simulink model "G474_Mode2_Direct_Start"  (R2024b)
settings: Solver=FixedStepDiscrete  StartTime=0.0  StopTime=q.stop_time  FixedStep=p.Ts  RelTol=1e-3
InitFcn:
  | m2_project_root=fileparts(fileparts(get_param(bdroot,'FileName')));Simulink.fileGenControl('set','CacheFolder',fullfile(m2_project_root,'work'),'CodeGenFolder',fullfile(m2_project_root,'work'),'createDir',true);
model workspace (MAT data in the model file):
  fSin = [0 0.00153398001567 0.00306795700453 0.00460192607716 0.00613588513806 0.00766982883215 0.00920375529677 0.0107376594096 0.0122715383768 0.0138053894043 0.0153392059729 0.0168729871511 ... (1025 elements, 1025x1)]
  p.Rs = 0.875
  p.Ls = 0.0002
  p.Ld = 0.0002
  p.Lq = 0.0002
  p.Flux = 0.00752
  p.MOTOR_POLES = 14
  p.Ts = 5e-05
  p.Gain = 5000
  p.PLL_BW_Hz = 15
  p.Comp_BW_Hz = 5
  p.PLL_kp = 188.495559215
  p.PLL_ki = 0.444132198049
  p.Comp_Kp = 62.8318530718
  p.Comp_Ki = 0.0493480220054
  p.Comp_Mode = 0
  p.SMO_Kslide = 10
  p.SMO_Boundary = 0.002
  p.V_deadtime = 0.3
  p.current_deadband = 0.01
  p.pll_step_limit = 0.157079632679
  p.speed_decimation = 8
  p.speed_filter_old = 0.95
  p.speed_filter_new = 0.05
  q.Ts = 5e-05
  q.Rs = 0.875
  q.Ld = 0.0002
  q.Lq = 0.0002
  q.Flux = 0.00752
  q.pole_pairs = 7
  q.target_rpm = 200
  q.second_rpm = 400
  q.third_rpm = 1000
  q.switch_1 = 0.8
  q.switch_2 = 1.6
  q.Vbus = 12
  q.stop_time = 4
  q.J = 2e-05
  q.B = 1e-05
  q.load_torque = 0.005
  q.initial_theta_e = 0.523598775598
  q.initial_rpm = 0
  q.actual_deadtime_V = 0.3
  q.speed_iq_sign = -1
  q.ramp_step = 0.05
  q.current_channel_sign = 1
  q.initial_state = [0; 0; 0; 0.523598775598]
  s0.psi_s = [0; 0]
  s0.theta = 0
(part 1 of 2)
settings Model: Creator=QXZ-030079  LastModifiedBy=QXZ-030079
settings DataIOCC: SignalLogging=off

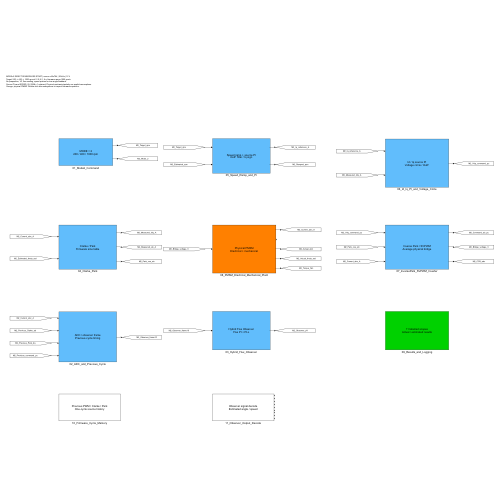
[thumbnail: Simulink's stored preview of the top-level diagram]
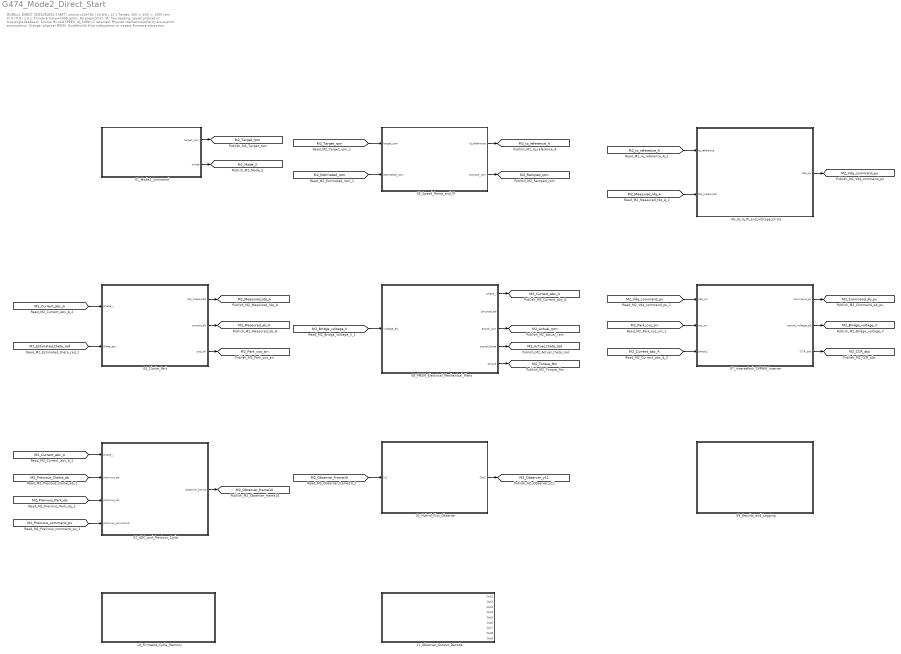
== system G474_Mode2_Direct_Start ==
  note: MODE=2 DIRECT SENSORLESS START | source c43e794 | 20 kHz | 12 V
      | Target: 200 -> 400 -> 1000 rpm at 0 / 0.8 / 1.6 s; firmware ramp=1000 rpm/s.
      | No preposition, VF, flux seeding, speed preload or true-angle feedback.
      | Source PIs and SPEED_IQ_SIGN=-1 retained. Physical mechanics/polarity are explicit assumptions.
      | Orange: physical PMSM. Double-click blue subsystems to inspect firmware equations.
  01_Mode2_Command : Subsystem
      mask Display: disp('MODE = 2\n200 / 400 / 1000 rpm');
  02_ADC_and_Previous_Cycle : Subsystem
      mask Display: disp('ADC / observer frame\nPrevious-cycle timing');
  03_Hybrid_Flux_Observer : Subsystem
      settings: OpenFcn=open_system(gcb,'force')
      mask Display: disp('Hybrid Flux Observer\nFlux PI + PLL');
  04_Clarke_Park : Subsystem
      mask Display: disp('Clarke / Park\nFirmware sine table');
  05_Speed_Ramp_and_PI : Subsystem
      mask Display: disp('Speed ramp + source PI\nOutF filter / Iq sign');
  06_Id_Iq_PI_and_Voltage_Circle : Subsystem
      mask Display: disp('Id / Iq source PI\nVoltage circle / OutF');
  07_InversePark_SVPWM_Inverter : Subsystem
      mask Display: disp('Inverse Park / SVPWM\nAverage physical bridge');
  08_PMSM_Electrical_Mechanical_Plant : Subsystem
      mask Display: disp('Physical PMSM\nElectrical + mechanical');
  09_Results_and_Logging : Subsystem
      mask Display: disp('11 labelled scopes\nActual / estimated results');
  10_Firmware_Cycle_Memory : Subsystem
      mask Display: disp('Previous PWM / Clarke / Park\nOne-cycle source history');
  11_Observer_Output_Decode : Subsystem
      mask Display: disp('Observer signal decode\nEstimated angle / speed');
  tag scope: M2_Actual_rpm=global, M2_Actual_theta_rad=global, M2_Bridge_voltage_V=global, M2_CCR_abc=global, M2_Command_ab_pu=global, M2_Current_abc_A=global, M2_Iq_reference_A=global, M2_Measured_Idq_A=global, M2_Measured_ab_A=global, M2_Mode_2=global, M2_Observer_frame10=global, M2_Observer_y11=global, M2_Park_cos_sin=global, M2_Ramped_rpm=global, M2_Target_rpm=global, M2_Torque_Nm=global, M2_Vdq_command_pu=global
  wires:
  01_Mode2_Command/2(mode) -> [M2_Mode_2]
  07_InversePark_SVPWM_Inverter/3(CCR_abc) -> [M2_CCR_abc]
  05_Speed_Ramp_and_PI/2(ramped_rpm) -> [M2_Ramped_rpm]
  08_PMSM_Electrical_Mechanical_Plant/5(torque) -> [M2_Torque_Nm]
  08_PMSM_Electrical_Mechanical_Plant/4(actual_theta) -> [M2_Actual_theta_rad]
  08_PMSM_Electrical_Mechanical_Plant/3(actual_rpm) -> [M2_Actual_rpm]
  07_InversePark_SVPWM_Inverter/2(actual_voltage_ab) -> [M2_Bridge_voltage_V]
  [M2_Bridge_voltage_V] -> 08_PMSM_Electrical_Mechanical_Plant/1(voltage_ab)
  04_Clarke_Park/3(cos_sin) -> [M2_Park_cos_sin]
  [M2_Park_cos_sin] -> 07_InversePark_SVPWM_Inverter/2(cos_sin)
  06_Id_Iq_PI_and_Voltage_Circle/1(Vdq_pu) -> [M2_Vdq_command_pu]
  [M2_Vdq_command_pu] -> 07_InversePark_SVPWM_Inverter/1(Vdq_pu)
  05_Speed_Ramp_and_PI/1(Iq_reference) -> [M2_Iq_reference_A]
  [M2_Iq_reference_A] -> 06_Id_Iq_PI_and_Voltage_Circle/1(Iq_reference)
  [M2_Estimated_rpm] -> 05_Speed_Ramp_and_PI/2(estimated_rpm)
  01_Mode2_Command/1(target_rpm) -> [M2_Target_rpm]
  [M2_Target_rpm] -> 05_Speed_Ramp_and_PI/1(target_rpm)
  [M2_Estimated_theta_rad] -> 04_Clarke_Park/2(theta_est)
  03_Hybrid_Flux_Observer/1(Out1) -> [M2_Observer_y11]
  02_ADC_and_Previous_Cycle/1(observer_frame) -> [M2_Observer_frame10]
  [M2_Observer_frame10] -> 03_Hybrid_Flux_Observer/1(In1)
  [M2_Previous_command_pu] -> 02_ADC_and_Previous_Cycle/4(previous_command)
  [M2_Previous_Park_dq] -> 02_ADC_and_Previous_Cycle/3(previous_dq)
  [M2_Previous_Clarke_ab] -> 02_ADC_and_Previous_Cycle/2(previous_ab)
  08_PMSM_Electrical_Mechanical_Plant/1(phase_i) -> [M2_Current_abc_A]
  [M2_Current_abc_A] -> 02_ADC_and_Previous_Cycle/1(phase_i)
  [M2_Current_abc_A] -> 04_Clarke_Park/1(phase_i)
  [M2_Current_abc_A] -> 07_InversePark_SVPWM_Inverter/3(phase_i)
  04_Clarke_Park/1(Idq_measured) -> [M2_Measured_Idq_A]
  [M2_Measured_Idq_A] -> 06_Id_Iq_PI_and_Voltage_Circle/2(Idq_measured)
  04_Clarke_Park/2(current_ab) -> [M2_Measured_ab_A]
  07_InversePark_SVPWM_Inverter/1(command_pu) -> [M2_Command_ab_pu]

== system G474_Mode2_Direct_Start/01_Mode2_Command ==
  Initial_200rpm : Constant  Value=q.target_rpm
  MODE_SENSORLESS_2 : Constant  Value=2
  Speed_schedule : Sum  Inputs=+++
  Switch_to_1000rpm : Step  Time=q.switch_2  After=q.third_rpm-q.second_rpm  SampleTime=p.Ts
  Switch_to_400rpm : Step  Time=q.switch_1  After=q.second_rpm-q.target_rpm  SampleTime=p.Ts
  target_rpm : Outport
  mode : Outport  Port=2
  wires:
  MODE_SENSORLESS_2/1 -> mode/1
  Speed_schedule/1 -> target_rpm/1
  Initial_200rpm/1 -> Speed_schedule/1
  Switch_to_400rpm/1 -> Speed_schedule/2
  Switch_to_1000rpm/1 -> Speed_schedule/3

== system G474_Mode2_Direct_Start/02_ADC_and_Previous_Cycle ==
  phase_i : Inport
  previous_ab : Inport  Port=2
  previous_dq : Inport  Port=3
  previous_command : Inport  Port=4
  Firmware_call_order : MATLAB Function  TreatAsAtomicUnit=on
  observer_frame : Outport
  wires:
  previous_command/1 -> Firmware_call_order/1(old_command)
  phase_i/1 -> Firmware_call_order/2(phase_i)
  previous_ab/1 -> Firmware_call_order/3(old_ab)
  previous_dq/1 -> Firmware_call_order/4(old_dq)
  Firmware_call_order/1(frame) -> observer_frame/1

== system G474_Mode2_Direct_Start/03_Hybrid_Flux_Observer ==
  In1 : Inport
  01_Voltage_Compensation : Subsystem
      settings: OpenFcn=open_system(gcb,'force')
      mask Display: port_label('input',1,'command_pu');port_label('input',2,'phase_current');port_label('input',3,'Vbus');port_label('input',4,'Km');port_label('output',1,'voltage_V');
  02_Active_Flux_Models : Subsystem
      settings: OpenFcn=open_system(gcb,'force')
      mask Display: port_label('input',1,'theta_previous');port_label('input',2,'current_ab');port_label('input',3,'psi_s_previous');port_label('input',4,'Id');port_label('output',1,'psi_I');port_label('output',2,'psi_V');
  03_Flux_Feedback : Subsystem
      settings: OpenFcn=open_system(gcb,'force')
      mask Display: port_label('input',1,'psi_I');port_label('input',2,'psi_V');port_label('output',1,'Ucomp');
  04_Stator_Integrator : Subsystem
      settings: OpenFcn=open_system(gcb,'force')
      mask Display: port_label('input',1,'voltage_V');port_label('input',2,'current_ab');port_label('input',3,'Ucomp');port_label('output',1,'psi_s_new');port_label('output',2,'psi_s_previous');
  05_PLL_and_Angle : Subsystem
      settings: OpenFcn=open_system(gcb,'force')
      mask Display: port_label('input',1,'psi_V');port_label('output',1,'theta_previous');port_label('output',2,'step_rad');port_label('output',3,'theta_new');port_label('output',4,'PLL_error');
  06_Speed_Filter : Subsystem
      settings: OpenFcn=open_system(gcb,'force')
      mask Display: port_label('input',1,'step_rad');port_label('output',1,'electrical_Hz');port_label('output',2,'firmware_RPM');
  Input split : Demux  Outputs=[2 3 2 1 1 1]
  Results : Mux  Inputs=8
  Out1 : Outport
  wires:
  03_Flux_Feedback/1(Ucomp) -> 04_Stator_Integrator/3(Ucomp)
  02_Active_Flux_Models/2(psi_V) -> 05_PLL_and_Angle/1(psi_V), Results/4, 03_Flux_Feedback/2(psi_V)
  06_Speed_Filter/2(firmware_RPM) -> Results/3
  06_Speed_Filter/1(electrical_Hz) -> Results/2
  Results/1 -> Out1/1
  04_Stator_Integrator/2(psi_s_previous) -> 02_Active_Flux_Models/3(psi_s_previous)
  04_Stator_Integrator/1(psi_s_new) -> Results/5
  05_PLL_and_Angle/4(PLL_error) -> Results/6
  05_PLL_and_Angle/3(theta_new) -> Results/1
  05_PLL_and_Angle/2(step_rad) -> 06_Speed_Filter/1(step_rad), Results/7
  01_Voltage_Compensation/1(voltage_V) -> 04_Stator_Integrator/1(voltage_V), Results/8
  Input split/5 -> 01_Voltage_Compensation/3(Vbus)
  02_Active_Flux_Models/1(psi_I) -> 03_Flux_Feedback/1(psi_I)
  Input split/6 -> 01_Voltage_Compensation/4(Km)
  Input split/3 -> 02_Active_Flux_Models/2(current_ab), 04_Stator_Integrator/2(current_ab)
  Input split/1 -> 01_Voltage_Compensation/1(command_pu)
  Input split/4 -> 02_Active_Flux_Models/4(Id)
  In1/1 -> Input split/1
  Input split/2 -> 01_Voltage_Compensation/2(phase_current)
  05_PLL_and_Angle/1(theta_previous) -> 02_Active_Flux_Models/1(theta_previous)

== system G474_Mode2_Direct_Start/04_Clarke_Park ==
  phase_i : Inport
  theta_est : Inport  Port=2
  Source_lookup_and_transform : MATLAB Function  TreatAsAtomicUnit=on
  Idq_measured : Outport
  current_ab : Outport  Port=2
  cos_sin : Outport  Port=3
  wires:
  phase_i/1 -> Source_lookup_and_transform/1(iabc)
  Source_lookup_and_transform/3(cs) -> cos_sin/1
  theta_est/1 -> Source_lookup_and_transform/2(theta)
  Source_lookup_and_transform/1(dq) -> Idq_measured/1
  Source_lookup_and_transform/2(iab) -> current_ab/1

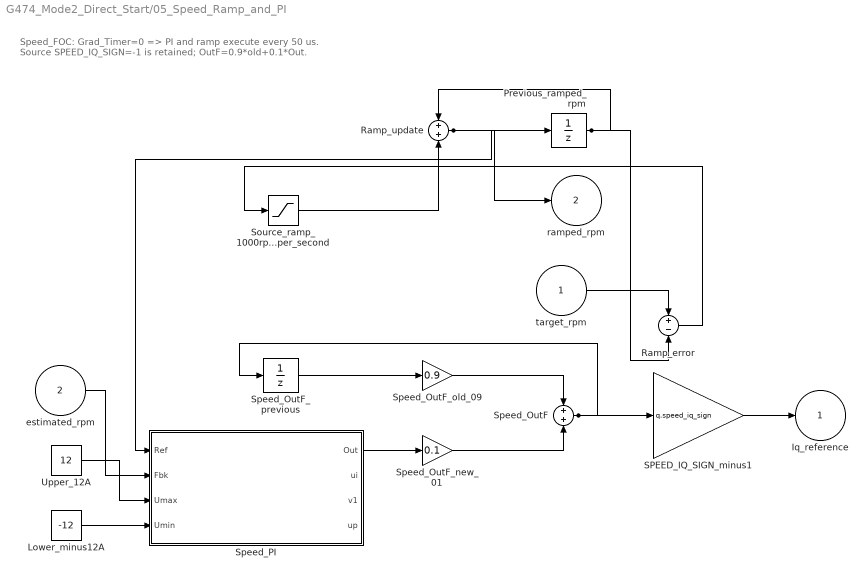
== system G474_Mode2_Direct_Start/05_Speed_Ramp_and_PI ==
  note: Speed_FOC: Grad_Timer=0 => PI and ramp execute every 50 us.
      | Source SPEED_IQ_SIGN=-1 is retained; OutF=0.9*old+0.1*Out.
  target_rpm : Inport
  estimated_rpm : Inport  Port=2
  Lower_minus12A : Constant  Value=-12
  Previous_ramped_rpm : UnitDelay  SampleTime=p.Ts  HasFrameUpgradeWarning=on
  Ramp_error : Sum  Inputs=+-
  Ramp_update : Sum
  SPEED_IQ_SIGN_minus1 : Gain  Gain=q.speed_iq_sign
  Source_ramp_1000rpm_per_second : Saturate  UpperLimit=q.ramp_step  LowerLimit=-q.ramp_step
  Speed_OutF : Sum
  Speed_OutF_new_01 : Gain  Gain=0.1
  Speed_OutF_old_09 : Gain  Gain=0.9
  Speed_OutF_previous : UnitDelay  SampleTime=p.Ts  HasFrameUpgradeWarning=on
  Speed_PI : Subsystem  mask{Kp=0.01, Ki=0.0001, Ts=p.Ts}
      mask prompts: Kp "Kp (source coefficient)"; Ki "Ki (per call, already discrete)"; Ts "Execution period (s)"
      settings: OpenFcn=open_system(gcb,'force')
      mask Display: port_label('input',1,'Ref');port_label('input',2,'Fbk');port_label('input',3,'Umax');port_label('input',4,'Umin');port_label('output',1,'Out');port_label('output',2,'ui');port_label('output',3,'v1');port_label('output',4,'up');
  Upper_12A : Constant  Value=12
  Iq_reference : Outport
  ramped_rpm : Outport  Port=2
  wires:
  Speed_OutF_old_09/1 -> Speed_OutF/1
  Ramp_update/1 -> Speed_PI/1(Ref), Previous_ramped_rpm/1, ramped_rpm/1
  Speed_PI/1(Out) -> Speed_OutF_new_01/1
  estimated_rpm/1 -> Speed_PI/2(Fbk)
  Upper_12A/1 -> Speed_PI/3(Umax)
  Source_ramp_1000rpm_per_second/1 -> Ramp_update/2
  Lower_minus12A/1 -> Speed_PI/4(Umin)
  Speed_OutF_previous/1 -> Speed_OutF_old_09/1
  target_rpm/1 -> Ramp_error/1
  Speed_OutF_new_01/1 -> Speed_OutF/2
  Previous_ramped_rpm/1 -> Ramp_error/2, Ramp_update/1
  Speed_OutF/1 -> Speed_OutF_previous/1, SPEED_IQ_SIGN_minus1/1
  Ramp_error/1 -> Source_ramp_1000rpm_per_second/1
  SPEED_IQ_SIGN_minus1/1 -> Iq_reference/1

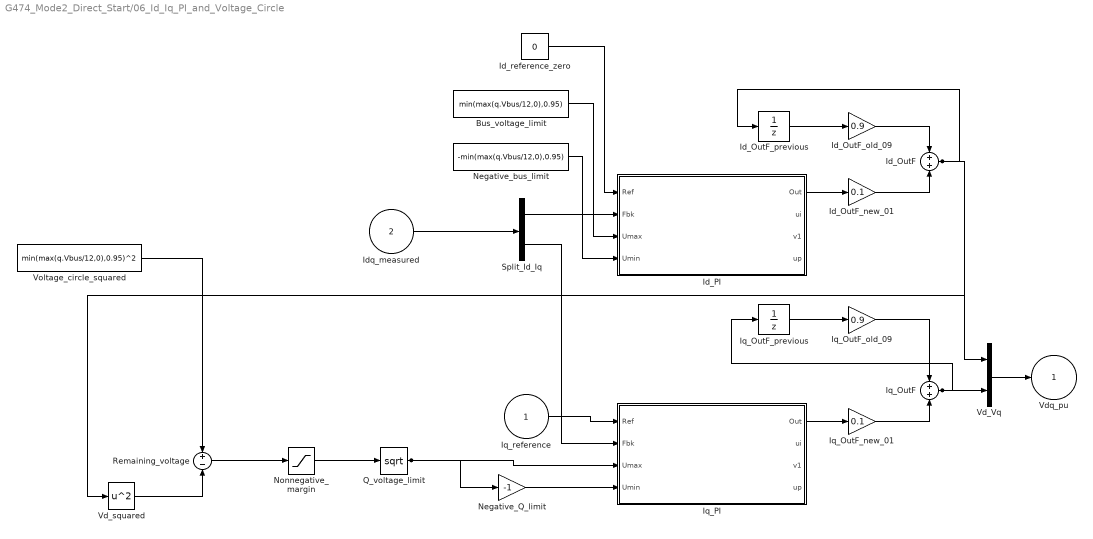
== system G474_Mode2_Direct_Start/06_Id_Iq_PI_and_Voltage_Circle ==
  Iq_reference : Inport
  Idq_measured : Inport  Port=2
  Bus_voltage_limit : Constant  Value=min(max(q.Vbus/12,0),0.95)
  Id_OutF : Sum
  Id_OutF_new_01 : Gain  Gain=0.1
  Id_OutF_old_09 : Gain  Gain=0.9
  Id_OutF_previous : UnitDelay  SampleTime=p.Ts  HasFrameUpgradeWarning=on
  Id_PI : Subsystem  mask{Kp=0.01, Ki=0.00001, Ts=p.Ts}
      mask prompts: Kp "Kp (source coefficient)"; Ki "Ki (per call, already discrete)"; Ts "Execution period (s)"
      settings: OpenFcn=open_system(gcb,'force')
      mask Display: port_label('input',1,'Ref');port_label('input',2,'Fbk');port_label('input',3,'Umax');port_label('input',4,'Umin');port_label('output',1,'Out');port_label('output',2,'ui');port_label('output',3,'v1');port_label('output',4,'up');
  Id_reference_zero : Constant  Value=0
  Iq_OutF : Sum
  Iq_OutF_new_01 : Gain  Gain=0.1
  Iq_OutF_old_09 : Gain  Gain=0.9
  Iq_OutF_previous : UnitDelay  SampleTime=p.Ts  HasFrameUpgradeWarning=on
  Iq_PI : Subsystem  mask{Kp=0.01, Ki=0.00001, Ts=p.Ts}
      mask prompts: Kp "Kp (source coefficient)"; Ki "Ki (per call, already discrete)"; Ts "Execution period (s)"
      settings: OpenFcn=open_system(gcb,'force')
      mask Display: port_label('input',1,'Ref');port_label('input',2,'Fbk');port_label('input',3,'Umax');port_label('input',4,'Umin');port_label('output',1,'Out');port_label('output',2,'ui');port_label('output',3,'v1');port_label('output',4,'up');
  Negative_Q_limit : Gain  Gain=-1
  Negative_bus_limit : Constant  Value=-min(max(q.Vbus/12,0),0.95)
  Nonnegative_margin : Saturate  UpperLimit=inf  LowerLimit=0
  Q_voltage_limit : Math  Operator=sqrt
  Remaining_voltage : Sum  Inputs=+-
  Split_Id_Iq : Demux  Outputs=2
  Vd_Vq : Mux  Inputs=2
  Vd_squared : Math  Operator=square
  Voltage_circle_squared : Constant  Value=min(max(q.Vbus/12,0),0.95)^2
  Vdq_pu : Outport
  wires:
  Id_reference_zero/1 -> Id_PI/1(Ref)
  Voltage_circle_squared/1 -> Remaining_voltage/1
  Remaining_voltage/1 -> Nonnegative_margin/1
  Iq_reference/1 -> Iq_PI/1(Ref)
  Vd_squared/1 -> Remaining_voltage/2
  Idq_measured/1 -> Split_Id_Iq/1
  Nonnegative_margin/1 -> Q_voltage_limit/1
  Q_voltage_limit/1 -> Iq_PI/3(Umax), Negative_Q_limit/1
  Bus_voltage_limit/1 -> Id_PI/3(Umax)
  Negative_bus_limit/1 -> Id_PI/4(Umin)
  Split_Id_Iq/1 -> Id_PI/2(Fbk)
  Split_Id_Iq/2 -> Iq_PI/2(Fbk)
  Negative_Q_limit/1 -> Iq_PI/4(Umin)
  Id_OutF_previous/1 -> Id_OutF_old_09/1
  Id_PI/1(Out) -> Id_OutF_new_01/1
  Iq_OutF_previous/1 -> Iq_OutF_old_09/1
  Iq_PI/1(Out) -> Iq_OutF_new_01/1
  Vd_Vq/1 -> Vdq_pu/1
  Id_OutF_old_09/1 -> Id_OutF/1
  Id_OutF_new_01/1 -> Id_OutF/2
  Iq_OutF_old_09/1 -> Iq_OutF/1
  Iq_OutF_new_01/1 -> Iq_OutF/2
  Id_OutF/1 -> Id_OutF_previous/1, Vd_squared/1, Vd_Vq/1
  Iq_OutF/1 -> Iq_OutF_previous/1, Vd_Vq/2

== system G474_Mode2_Direct_Start/07_InversePark_SVPWM_Inverter ==
  note: Source SVPWM sector / CCR truncation / 0..3999 clamp retained.
      | Plant voltage is reconstructed from duty ratios, not forced to observer voltage.
  Vdq_pu : Inport
  cos_sin : Inport  Port=2
  phase_i : Inport  Port=3
  Inverse_Park : MATLAB Function  TreatAsAtomicUnit=on
  Source_SVPWM_and_average_bridge : MATLAB Function  TreatAsAtomicUnit=on
  command_pu : Outport
  actual_voltage_ab : Outport  Port=2
  CCR_abc : Outport  Port=3
  wires:
  Inverse_Park/1(command) -> command_pu/1, Source_SVPWM_and_average_bridge/1(command)
  Vdq_pu/1 -> Inverse_Park/1(vdq)
  cos_sin/1 -> Inverse_Park/2(cs)
  phase_i/1 -> Source_SVPWM_and_average_bridge/2(iabc)
  Source_SVPWM_and_average_bridge/1(voltage) -> actual_voltage_ab/1
  Source_SVPWM_and_average_bridge/2(ccr) -> CCR_abc/1

== system G474_Mode2_Direct_Start/08_PMSM_Electrical_Mechanical_Plant ==
  note: True angle/speed are used only by the physical plant and result plots.
      | J=2e-5 kg*m^2, B=1e-5 N*m*s/rad, load=0.005 N*m: assumed, adjustable.
      | Initial speed/current=0; initial electrical angle=30 deg; observer state=0.
  voltage_ab : Inport
  Electrical_and_mechanical_RK4 : MATLAB Function  TreatAsAtomicUnit=on
  Physical_measurements : MATLAB Function  TreatAsAtomicUnit=on
  Physical_state_id_iq_wm_theta : UnitDelay  InitialCondition=q.initial_state  SampleTime=p.Ts  HasFrameUpgradeWarning=on
  phase_i : Outport
  physical_ab : Outport  Port=2
  actual_rpm : Outport  Port=3
  actual_theta : Outport  Port=4
  torque : Outport  Port=5
  wires:
  Electrical_and_mechanical_RK4/1(xn) -> Physical_state_id_iq_wm_theta/1
  Physical_state_id_iq_wm_theta/1 -> Electrical_and_mechanical_RK4/1(x), Physical_measurements/1(x)
  voltage_ab/1 -> Electrical_and_mechanical_RK4/2(v)
  Physical_measurements/1(iabc) -> phase_i/1
  Physical_measurements/2(iab) -> physical_ab/1
  Physical_measurements/3(rpm) -> actual_rpm/1
  Physical_measurements/4(theta) -> actual_theta/1
  Physical_measurements/5(torque) -> torque/1

== system G474_Mode2_Direct_Start/09_Results_and_Logging ==
  09_Results_11_Scopes : Subsystem
  Logging_taps : Subsystem
  tag scope: M2_Full_log34=global
  wires:
  [M2_Full_log34] -> 09_Results_11_Scopes/1(signals34)
  Logging_taps/1(Out1) -> [M2_Full_log34]

== system G474_Mode2_Direct_Start/10_Firmware_Cycle_Memory ==
  Previous_Clarke_ab : UnitDelay  InitialCondition=[0;0]  SampleTime=p.Ts  HasFrameUpgradeWarning=on
  Previous_Park_dq : UnitDelay  InitialCondition=[0;0]  SampleTime=p.Ts  HasFrameUpgradeWarning=on
  Previous_command_pu : UnitDelay  InitialCondition=[0;0]  SampleTime=p.Ts  HasFrameUpgradeWarning=on
  tag scope: M2_Previous_Clarke_ab=global, M2_Previous_Park_dq=global, M2_Previous_command_pu=global
  wires:
  [M2_Measured_ab_A] -> Previous_Clarke_ab/1
  [M2_Command_ab_pu] -> Previous_command_pu/1
  Previous_Park_dq/1 -> [M2_Previous_Park_dq]
  [M2_Measured_Idq_A] -> Previous_Park_dq/1
  Previous_Clarke_ab/1 -> [M2_Previous_Clarke_ab]
  Previous_command_pu/1 -> [M2_Previous_command_pu]

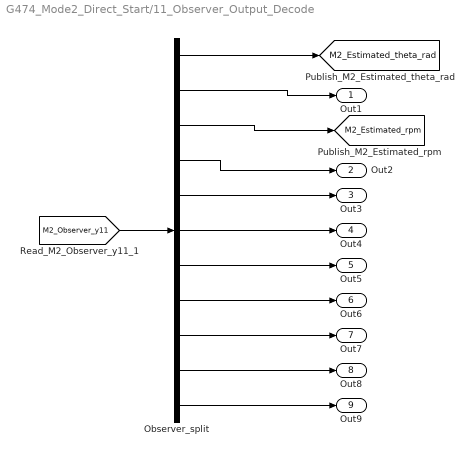
== system G474_Mode2_Direct_Start/11_Observer_Output_Decode ==
  Observer_split : Demux  Outputs=11
  Out1 : Outport
  Out2 : Outport  Port=2
  Out3 : Outport  Port=3
  Out4 : Outport  Port=4
  Out5 : Outport  Port=5
  Out6 : Outport  Port=6
  Out7 : Outport  Port=7
  Out8 : Outport  Port=8
  Out9 : Outport  Port=9
  tag scope: M2_Estimated_rpm=global, M2_Estimated_theta_rad=global
  wires:
  Observer_split/1 -> [M2_Estimated_theta_rad]
  [M2_Observer_y11] -> Observer_split/1
  Observer_split/2 -> Out1/1
  Observer_split/3 -> [M2_Estimated_rpm]
  Observer_split/4 -> Out2/1
  Observer_split/5 -> Out3/1
  Observer_split/6 -> Out4/1
  Observer_split/7 -> Out5/1
  Observer_split/8 -> Out6/1
  Observer_split/9 -> Out7/1
  Observer_split/10 -> Out8/1
  Observer_split/11 -> Out9/1

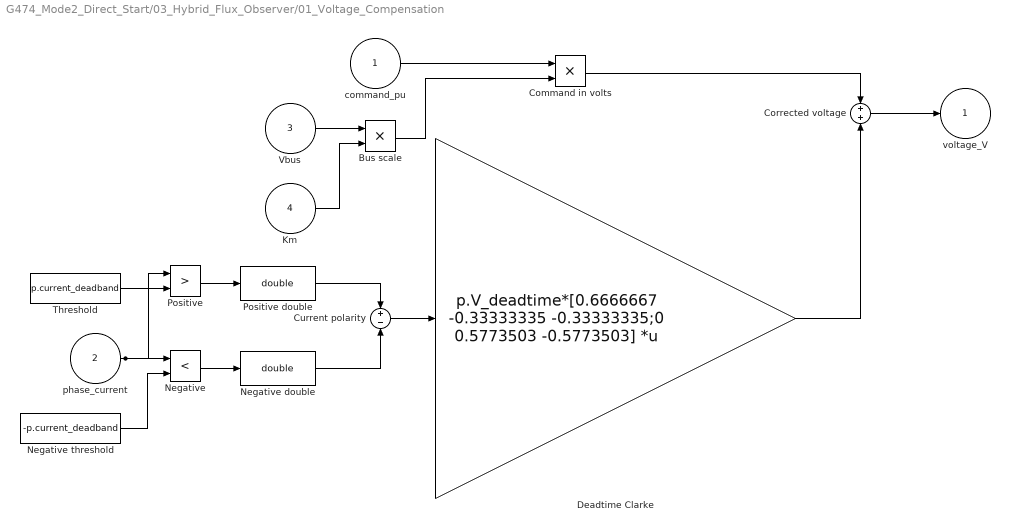
== system G474_Mode2_Direct_Start/03_Hybrid_Flux_Observer/01_Voltage_Compensation ==
  command_pu : Inport
  phase_current : Inport  Port=2
  Vbus : Inport  Port=3
  Km : Inport  Port=4
  Bus scale : Product  Inputs=**
  Command in volts : Product  Inputs=**
  Corrected voltage : Sum
  Current polarity : Sum  Inputs=+-
  Deadtime Clarke : Gain  Gain=p.V_deadtime*[0.6666667 -0.33333335 -0.33333335;0 0.5773503 -0.5773503]  Multiplication=Matrix(K*u)
  Negative : RelationalOperator  Operator=<  OutDataTypeStr=boolean  RndMeth=Simplest  InputSameDT=off
  Negative double : DataTypeConversion  OutDataTypeStr=double  SaturateOnIntegerOverflow=off  RndMeth=Floor
  Negative threshold : Constant  Value=-p.current_deadband
  Positive : RelationalOperator  Operator=>  OutDataTypeStr=boolean  RndMeth=Simplest  InputSameDT=off
  Positive double : DataTypeConversion  OutDataTypeStr=double  SaturateOnIntegerOverflow=off  RndMeth=Floor
  Threshold : Constant  Value=p.current_deadband
  voltage_V : Outport
  wires:
  Corrected voltage/1 -> voltage_V/1
  Deadtime Clarke/1 -> Corrected voltage/2
  Command in volts/1 -> Corrected voltage/1
  Current polarity/1 -> Deadtime Clarke/1
  Bus scale/1 -> Command in volts/2
  command_pu/1 -> Command in volts/1
  Vbus/1 -> Bus scale/1
  Negative double/1 -> Current polarity/2
  Negative/1 -> Negative double/1
  Positive double/1 -> Current polarity/1
  Negative threshold/1 -> Negative/2
  Km/1 -> Bus scale/2
  phase_current/1 -> Negative/1, Positive/1
  Positive/1 -> Positive double/1
  Threshold/1 -> Positive/2

== system G474_Mode2_Direct_Start/03_Hybrid_Flux_Observer/02_Active_Flux_Models ==
  theta_previous : Inport
  current_ab : Inport  Port=2
  psi_s_previous : Inport  Port=3
  Id : Inport  Port=4
  Current model : Subsystem
      settings: OpenFcn=open_system(gcb,'force')
      mask Display: port_label('input',1,'theta_previous');port_label('input',2,'Id');port_label('output',1,'psi_I');
  Voltage model extraction : Subsystem
      settings: OpenFcn=open_system(gcb,'force')
      mask Display: port_label('input',1,'psi_s_previous');port_label('input',2,'current_ab');port_label('output',1,'psi_V');
  psi_I : Outport
  psi_V : Outport  Port=2
  wires:
  psi_s_previous/1 -> Voltage model extraction/1(psi_s_previous)
  Current model/1(psi_I) -> psi_I/1
  current_ab/1 -> Voltage model extraction/2(current_ab)
  Id/1 -> Current model/2(Id)
  Voltage model extraction/1(psi_V) -> psi_V/1
  theta_previous/1 -> Current model/1(theta_previous)

== system G474_Mode2_Direct_Start/03_Hybrid_Flux_Observer/03_Flux_Feedback ==
  psi_I : Inport
  psi_V : Inport  Port=2
  Alpha beta errors : Demux  Outputs=2
  Alpha_PI : Subsystem  mask{Kp=p.Comp_Kp, Ki=p.Comp_Ki, Ts=p.Ts}
      mask prompts: Kp "Kp (source coefficient)"; Ki "Ki (per call, already discrete)"; Ts "Execution period (s)"
      settings: OpenFcn=open_system(gcb,'force')
      mask Display: port_label('input',1,'error');port_label('input',2,'integral_enable');port_label('output',1,'Ucomp');port_label('output',2,'integral');
  Beta_PI : Subsystem  mask{Kp=p.Comp_Kp, Ki=p.Comp_Ki, Ts=p.Ts}
      mask prompts: Kp "Kp (source coefficient)"; Ki "Ki (per call, already discrete)"; Ts "Execution period (s)"
      settings: OpenFcn=open_system(gcb,'force')
      mask Display: port_label('input',1,'error');port_label('input',2,'integral_enable');port_label('output',1,'Ucomp');port_label('output',2,'integral');
  Compensation mode : Constant  Value=p.Comp_Mode
  Flux error : Sum  Inputs=+-
  PI enable : Constant  Value=p.Comp_Mode==0
  PI voltage : Mux  Inputs=2
  SMO_feedback : Subsystem
      settings: OpenFcn=open_system(gcb,'force')
      mask Display: port_label('input',1,'In1');port_label('output',1,'Out1');
  Select feedback : Switch  Criteria=u2 ~= 0  SaturateOnIntegerOverflow=off  InputSameDT=off
  Ucomp : Outport
  wires:
  Select feedback/1 -> Ucomp/1
  Compensation mode/1 -> Select feedback/2
  Beta_PI/1(Ucomp) -> PI voltage/2
  Alpha_PI/1(Ucomp) -> PI voltage/1
  SMO_feedback/1(Out1) -> Select feedback/1
  PI enable/1 -> Beta_PI/2(integral_enable), Alpha_PI/2(integral_enable)
  Alpha beta errors/2 -> Beta_PI/1(error)
  psi_V/1 -> Flux error/2
  Flux error/1 -> Alpha beta errors/1, SMO_feedback/1(In1)
  psi_I/1 -> Flux error/1
  PI voltage/1 -> Select feedback/3
  Alpha beta errors/1 -> Alpha_PI/1(error)

== system G474_Mode2_Direct_Start/03_Hybrid_Flux_Observer/04_Stator_Integrator ==
  voltage_V : Inport
  current_ab : Inport  Port=2
  Ucomp : Inport  Port=3
  Euler Ts : Gain  Gain=p.Ts
  Flux derivative : Sum  Inputs=+-+
  Resistive voltage : Gain  Gain=p.Rs
  Stator memory : UnitDelay  InitialCondition=s0.psi_s  SampleTime=p.Ts  HasFrameUpgradeWarning=on
  Updated flux : Sum
  psi_s_new : Outport
  psi_s_previous : Outport  Port=2
  wires:
  Euler Ts/1 -> Updated flux/2
  Updated flux/1 -> Stator memory/1, psi_s_new/1
  Flux derivative/1 -> Euler Ts/1
  Resistive voltage/1 -> Flux derivative/2
  Stator memory/1 -> psi_s_previous/1, Updated flux/1
  voltage_V/1 -> Flux derivative/1
  Ucomp/1 -> Flux derivative/3
  current_ab/1 -> Resistive voltage/1

== system G474_Mode2_Direct_Start/03_Hybrid_Flux_Observer/05_PLL_and_Angle ==
  psi_V : Inport
  PLL : Subsystem
      settings: OpenFcn=open_system(gcb,'force')
      mask Display: port_label('input',1,'psi_V');port_label('input',2,'theta_previous');port_label('output',1,'theta_new');port_label('output',2,'step_rad');port_label('output',3,'PLL_error');
  Previous PLL angle : UnitDelay  InitialCondition=s0.theta  SampleTime=p.Ts  HasFrameUpgradeWarning=on
  theta_previous : Outport
  step_rad : Outport  Port=2
  theta_new : Outport  Port=3
  PLL_error : Outport  Port=4
  wires:
  PLL/2(step_rad) -> step_rad/1
  psi_V/1 -> PLL/1(psi_V)
  PLL/1(theta_new) -> theta_new/1, Previous PLL angle/1
  Previous PLL angle/1 -> theta_previous/1, PLL/2(theta_previous)
  PLL/3(PLL_error) -> PLL_error/1

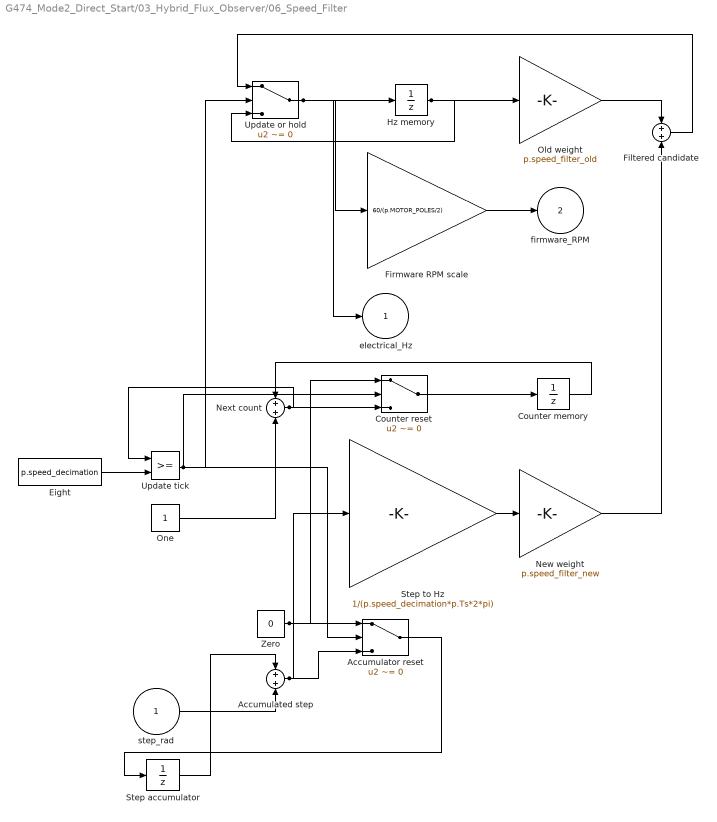
== system G474_Mode2_Direct_Start/03_Hybrid_Flux_Observer/06_Speed_Filter ==
  step_rad : Inport
  Accumulated step : Sum
  Accumulator reset : Switch  Criteria=u2 ~= 0  SaturateOnIntegerOverflow=off  InputSameDT=off
  Counter memory : UnitDelay  SampleTime=p.Ts  HasFrameUpgradeWarning=on
  Counter reset : Switch  Criteria=u2 ~= 0  SaturateOnIntegerOverflow=off  InputSameDT=off
  Eight : Constant  Value=p.speed_decimation
  Filtered candidate : Sum
  Firmware RPM scale : Gain  Gain=60/(p.MOTOR_POLES/2)
  Hz memory : UnitDelay  SampleTime=p.Ts  HasFrameUpgradeWarning=on
  New weight : Gain  Gain=p.speed_filter_new
  Next count : Sum
  Old weight : Gain  Gain=p.speed_filter_old
  One : Constant
  Step accumulator : UnitDelay  SampleTime=p.Ts  HasFrameUpgradeWarning=on
  Step to Hz : Gain  Gain=1/(p.speed_decimation*p.Ts*2*pi)
  Update or hold : Switch  Criteria=u2 ~= 0  SaturateOnIntegerOverflow=off  InputSameDT=off
  Update tick : RelationalOperator  OutDataTypeStr=boolean  RndMeth=Simplest  InputSameDT=off
  Zero : Constant  Value=0
  electrical_Hz : Outport
  firmware_RPM : Outport  Port=2
  wires:
  Filtered candidate/1 -> Update or hold/1
  New weight/1 -> Filtered candidate/2
  Counter memory/1 -> Next count/1
  Old weight/1 -> Filtered candidate/1
  Counter reset/1 -> Counter memory/1
  Hz memory/1 -> Old weight/1, Update or hold/3
  Accumulated step/1 -> Step to Hz/1, Accumulator reset/3
  Update or hold/1 -> Firmware RPM scale/1, electrical_Hz/1, Hz memory/1
  Step to Hz/1 -> New weight/1
  Step accumulator/1 -> Accumulated step/1
  step_rad/1 -> Accumulated step/2
  Firmware RPM scale/1 -> firmware_RPM/1
  Update tick/1 -> Update or hold/2, Accumulator reset/2, Counter reset/2
  Next count/1 -> Update tick/1, Counter reset/3
  Eight/1 -> Update tick/2
  One/1 -> Next count/2
  Zero/1 -> Accumulator reset/1, Counter reset/1
  Accumulator reset/1 -> Step accumulator/1

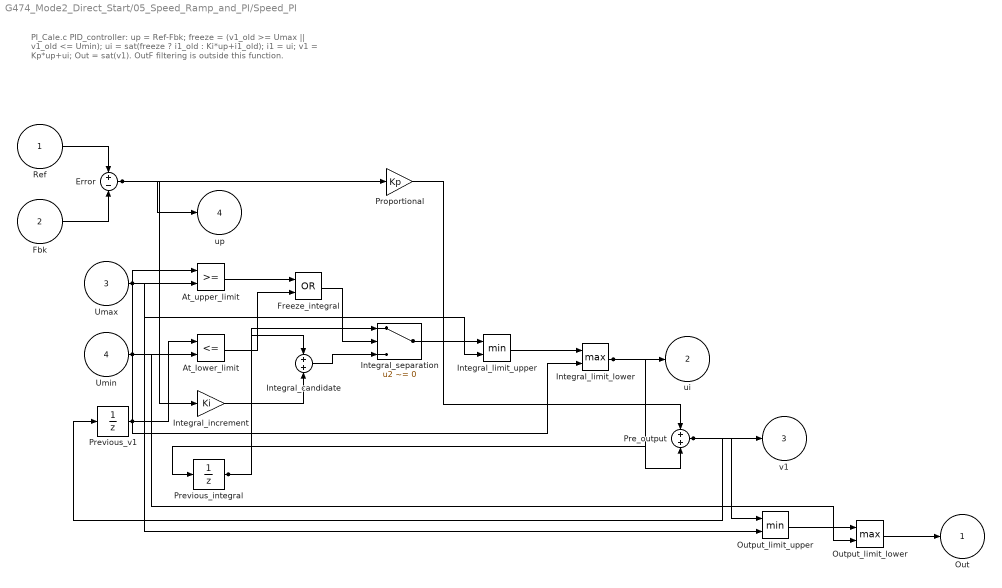
== system G474_Mode2_Direct_Start/05_Speed_Ramp_and_PI/Speed_PI ==
  note: PI_Cale.c PID_controller:
      | up = Ref-Fbk; freeze = (v1_old >= Umax || v1_old <= Umin);
      | ui = sat(freeze ? i1_old : Ki*up+i1_old); i1 = ui;
      | v1 = Kp*up+ui; Out = sat(v1). OutF filtering is outside this function.
  Ref : Inport
  Fbk : Inport  Port=2
  Umax : Inport  Port=3
  Umin : Inport  Port=4
  At_lower_limit : RelationalOperator  Operator=<=  OutDataTypeStr=boolean  RndMeth=Simplest  InputSameDT=off
  At_upper_limit : RelationalOperator  OutDataTypeStr=boolean  RndMeth=Simplest  InputSameDT=off
  Error : Sum  Inputs=+-
  Freeze_integral : Logic  Operator=OR  AllPortsSameDT=off  OutDataTypeStr=boolean
  Integral_candidate : Sum
  Integral_increment : Gain  Gain=Ki
  Integral_limit_lower : MinMax  Function=max  Inputs=2
  Integral_limit_upper : MinMax  Inputs=2
  Integral_separation : Switch  Criteria=u2 ~= 0  SaturateOnIntegerOverflow=off  InputSameDT=off
  Output_limit_lower : MinMax  Function=max  Inputs=2
  Output_limit_upper : MinMax  Inputs=2
  Pre_output : Sum
  Previous_integral : UnitDelay  SampleTime=Ts  HasFrameUpgradeWarning=on
  Previous_v1 : UnitDelay  SampleTime=Ts  HasFrameUpgradeWarning=on
  Proportional : Gain  Gain=Kp
  Out : Outport
  ui : Outport  Port=2
  v1 : Outport  Port=3
  up : Outport  Port=4
  wires:
  Previous_v1/1 -> At_upper_limit/1, At_lower_limit/1
  Umax/1 -> Output_limit_upper/2, At_upper_limit/2, Integral_limit_upper/2
  Ref/1 -> Error/1
  At_lower_limit/1 -> Freeze_integral/2
  Error/1 -> Proportional/1, Integral_increment/1, up/1
  Fbk/1 -> Error/2
  At_upper_limit/1 -> Freeze_integral/1
  Umin/1 -> Integral_limit_lower/2, Output_limit_lower/2, At_lower_limit/2
  Integral_increment/1 -> Integral_candidate/2
  Previous_integral/1 -> Integral_candidate/1, Integral_separation/1
  Freeze_integral/1 -> Integral_separation/2
  Integral_candidate/1 -> Integral_separation/3
  Proportional/1 -> Pre_output/1
  Integral_separation/1 -> Integral_limit_upper/1
  Integral_limit_upper/1 -> Integral_limit_lower/1
  Integral_limit_lower/1 -> Previous_integral/1, Pre_output/2, ui/1
  Pre_output/1 -> Previous_v1/1, Output_limit_upper/1, v1/1
  Output_limit_upper/1 -> Output_limit_lower/1
  Output_limit_lower/1 -> Out/1

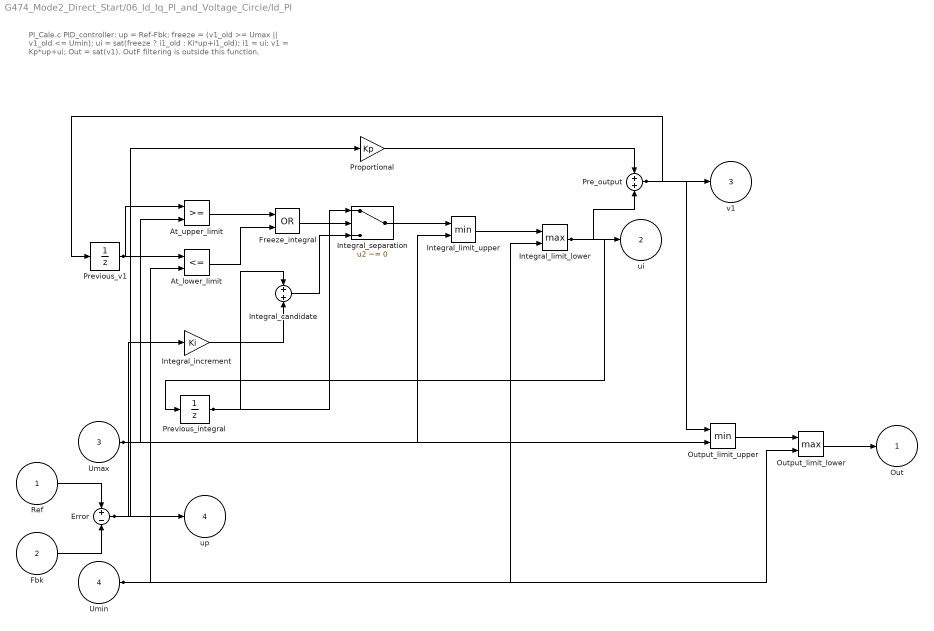
== system G474_Mode2_Direct_Start/06_Id_Iq_PI_and_Voltage_Circle/Id_PI ==
  note: PI_Cale.c PID_controller:
      | up = Ref-Fbk; freeze = (v1_old >= Umax || v1_old <= Umin);
      | ui = sat(freeze ? i1_old : Ki*up+i1_old); i1 = ui;
      | v1 = Kp*up+ui; Out = sat(v1). OutF filtering is outside this function.
  Ref : Inport
  Fbk : Inport  Port=2
  Umax : Inport  Port=3
  Umin : Inport  Port=4
  At_lower_limit : RelationalOperator  Operator=<=  OutDataTypeStr=boolean  RndMeth=Simplest  InputSameDT=off
  At_upper_limit : RelationalOperator  OutDataTypeStr=boolean  RndMeth=Simplest  InputSameDT=off
  Error : Sum  Inputs=+-
  Freeze_integral : Logic  Operator=OR  AllPortsSameDT=off  OutDataTypeStr=boolean
  Integral_candidate : Sum
  Integral_increment : Gain  Gain=Ki
  Integral_limit_lower : MinMax  Function=max  Inputs=2
  Integral_limit_upper : MinMax  Inputs=2
  Integral_separation : Switch  Criteria=u2 ~= 0  SaturateOnIntegerOverflow=off  InputSameDT=off
  Output_limit_lower : MinMax  Function=max  Inputs=2
  Output_limit_upper : MinMax  Inputs=2
  Pre_output : Sum
  Previous_integral : UnitDelay  SampleTime=Ts  HasFrameUpgradeWarning=on
  Previous_v1 : UnitDelay  SampleTime=Ts  HasFrameUpgradeWarning=on
  Proportional : Gain  Gain=Kp
  Out : Outport
  ui : Outport  Port=2
  v1 : Outport  Port=3
  up : Outport  Port=4
  wires:
  Umax/1 -> Output_limit_upper/2, Integral_limit_upper/2, At_upper_limit/2
  Previous_v1/1 -> At_upper_limit/1, At_lower_limit/1
  Ref/1 -> Error/1
  At_lower_limit/1 -> Freeze_integral/2
  Error/1 -> Proportional/1, Integral_increment/1, up/1
  Fbk/1 -> Error/2
  At_upper_limit/1 -> Freeze_integral/1
  Umin/1 -> Integral_limit_lower/2, Output_limit_lower/2, At_lower_limit/2
  Integral_increment/1 -> Integral_candidate/2
  Previous_integral/1 -> Integral_candidate/1, Integral_separation/1
  Freeze_integral/1 -> Integral_separation/2
  Integral_candidate/1 -> Integral_separation/3
  Proportional/1 -> Pre_output/1
  Integral_separation/1 -> Integral_limit_upper/1
  Integral_limit_upper/1 -> Integral_limit_lower/1
  Integral_limit_lower/1 -> Pre_output/2, Previous_integral/1, ui/1
  Pre_output/1 -> Previous_v1/1, Output_limit_upper/1, v1/1
  Output_limit_upper/1 -> Output_limit_lower/1
  Output_limit_lower/1 -> Out/1

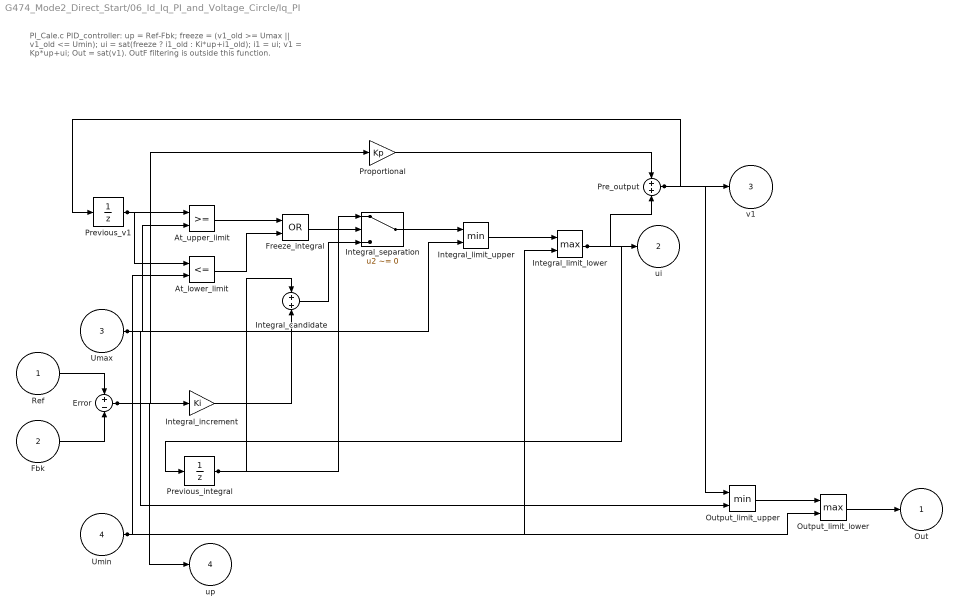
== system G474_Mode2_Direct_Start/06_Id_Iq_PI_and_Voltage_Circle/Iq_PI ==
  note: PI_Cale.c PID_controller:
      | up = Ref-Fbk; freeze = (v1_old >= Umax || v1_old <= Umin);
      | ui = sat(freeze ? i1_old : Ki*up+i1_old); i1 = ui;
      | v1 = Kp*up+ui; Out = sat(v1). OutF filtering is outside this function.
  Ref : Inport
  Fbk : Inport  Port=2
  Umax : Inport  Port=3
  Umin : Inport  Port=4
  At_lower_limit : RelationalOperator  Operator=<=  OutDataTypeStr=boolean  RndMeth=Simplest  InputSameDT=off
  At_upper_limit : RelationalOperator  OutDataTypeStr=boolean  RndMeth=Simplest  InputSameDT=off
  Error : Sum  Inputs=+-
  Freeze_integral : Logic  Operator=OR  AllPortsSameDT=off  OutDataTypeStr=boolean
  Integral_candidate : Sum
  Integral_increment : Gain  Gain=Ki
  Integral_limit_lower : MinMax  Function=max  Inputs=2
  Integral_limit_upper : MinMax  Inputs=2
  Integral_separation : Switch  Criteria=u2 ~= 0  SaturateOnIntegerOverflow=off  InputSameDT=off
  Output_limit_lower : MinMax  Function=max  Inputs=2
  Output_limit_upper : MinMax  Inputs=2
  Pre_output : Sum
  Previous_integral : UnitDelay  SampleTime=Ts  HasFrameUpgradeWarning=on
  Previous_v1 : UnitDelay  SampleTime=Ts  HasFrameUpgradeWarning=on
  Proportional : Gain  Gain=Kp
  Out : Outport
  ui : Outport  Port=2
  v1 : Outport  Port=3
  up : Outport  Port=4
  wires:
  Umax/1 -> Output_limit_upper/2, Integral_limit_upper/2, At_upper_limit/2
  Ref/1 -> Error/1
  At_lower_limit/1 -> Freeze_integral/2
  Error/1 -> Proportional/1, Integral_increment/1, up/1
  Fbk/1 -> Error/2
  Previous_v1/1 -> At_lower_limit/1, At_upper_limit/1
  At_upper_limit/1 -> Freeze_integral/1
  Umin/1 -> Integral_limit_lower/2, Output_limit_lower/2, At_lower_limit/2
  Integral_increment/1 -> Integral_candidate/2
  Integral_separation/1 -> Integral_limit_upper/1
  Previous_integral/1 -> Integral_candidate/1, Integral_separation/1
  Freeze_integral/1 -> Integral_separation/2
  Integral_candidate/1 -> Integral_separation/3
  Proportional/1 -> Pre_output/1
  Integral_limit_upper/1 -> Integral_limit_lower/1
  Integral_limit_lower/1 -> Previous_integral/1, Pre_output/2, ui/1
  Pre_output/1 -> Previous_v1/1, Output_limit_upper/1, v1/1
  Output_limit_upper/1 -> Output_limit_lower/1
  Output_limit_lower/1 -> Out/1
